simulink model "jaka_fk_exp"  (R2022b)
settings: Solver=FixedStepAuto  StartTime=0.0  StopTime=10.0  RelTol=1e-3
model workspace (MAT data in the model file):
  SL_ROS_VariableLengthArrays_MaxSizes.CommonInfo.ArrayTruncateAction = 'EmitWarning'
  SL_ROS_VariableLengthArrays_MaxSizes.MsgTypeMap = containers.Map
  SL_ROS_VariableLengthArrays_MaxSizes.MsgTypeMap.serialization.keys = {'jaka_msgs/MoveRequest'}
  SL_ROS_VariableLengthArrays_MaxSizes.MsgTypeMap.serialization.values{1}(1).PropertyName = 'Pose'
  SL_ROS_VariableLengthArrays_MaxSizes.MsgTypeMap.serialization.values{1}(1).DataType = 'single'
  SL_ROS_VariableLengthArrays_MaxSizes.MsgTypeMap.serialization.values{1}(1).MaxLength = 6
  SL_ROS_VariableLengthArrays_MaxSizes.MsgTypeMap.serialization.values{1}(2).PropertyName = 'RefJoint'
  SL_ROS_VariableLengthArrays_MaxSizes.MsgTypeMap.serialization.values{1}(2).DataType = 'single'
  SL_ROS_VariableLengthArrays_MaxSizes.MsgTypeMap.serialization.values{1}(2).MaxLength = 6
  SL_ROS_VariableLengthArrays_MaxSizes.MsgTypeMap.serialization.uniformity = 0
  SL_ROS_VariableLengthArrays_MaxSizes.MsgTypeMap.serialization.keyType = 'char'
  SL_ROS_VariableLengthArrays_MaxSizes.MsgTypeMap.serialization.valueType = 'any'
undefined symbols (not defined in the file or in its folder): Mvacc, Mvvelo, Pose, Pose_SL_Info
libraries: robotlib x2
settings Model: Creator=boen  LastModifiedBy=boen
settings OptimizationCC: EnhancedBackFolding=on  PassReuseOutputArgsAs=Individual arguments  ZeroExternalMemoryAtStartup=off  ZeroInternalMemoryAtStartup=off  MaxStackSize=64  OptimizeBlockOrder=speed  DifferentSizesBufferReuse=on  OptimizationCustomize=off  EfficientTunableParamExpr=on
settings DebuggingCC: ParameterTunabilityLossMsg=error
settings HardwareCC: ProdBitPerLong=64  ProdLargestAtomicInteger=LongLong  ProdLargestAtomicFloat=Double  ProdLongLongMode=on  ProdHWDeviceType=ARM Compatible->ARM 64-bit (LP64)
settings SFSimCC: MATLABDynamicMemAlloc=off
settings RTWCC: Description=Embedded Coder  SystemTargetFile=ert.tlc  HardwareBoard=Robot Operating System (ROS)  TLCOptions="-aInlineSetEventsForThisBaseRateFcn=TLC_FALSE -aSuppressMultiTaskScheduler=TLC_FALSE  -aRateBasedStepFcn=0"  TemplateMakefile=ert_default_tmf  Toolchain=Catkin  TargetLang=C++
settings CodeAppCC: ForceParamTrailComments=on  IgnoreCustomStorageClasses=off  OperatorAnnotations=on  SimulinkDataObjDesc=on  SFDataObjDesc=on  InsertBlockDesc=on

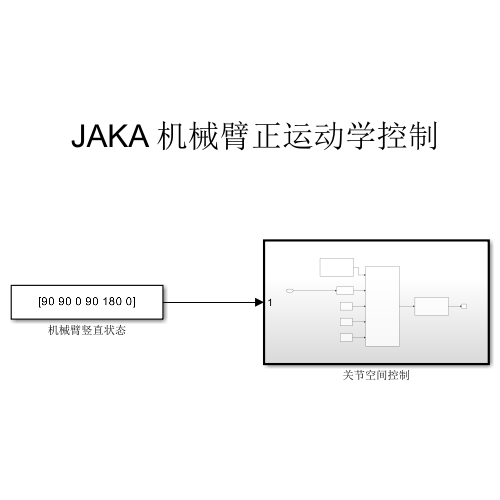
[thumbnail: Simulink's stored preview of the top-level diagram]
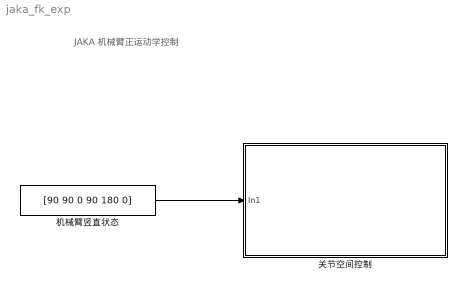
== system jaka_fk_exp ==
  note: JAKA 机械臂正运动学控制
  关节空间控制 : Subsystem  TreatAsAtomicUnit=on
  机械臂竖直状态 : Constant  Value=[90 90 0 90 180 0]
  wires:
  机械臂竖直状态/1 -> 关节空间控制/1(In1)

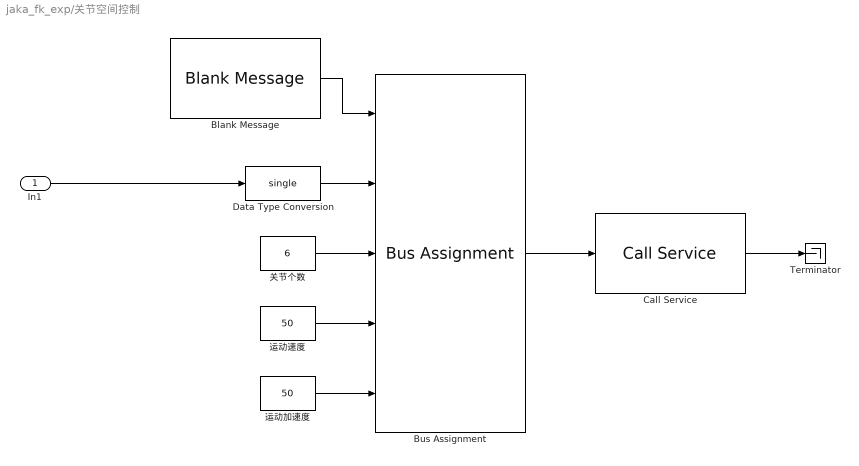
== system jaka_fk_exp/关节空间控制 ==
  In1 : Inport
  Blank Message : robotlib/Blank Message  messageClass=Service Request  entityType=jaka_msgs/Move  messageType=jaka_msgs/MoveRequest  SampleTime=inf  legacyBusStruct=off
  Bus Assignment : BusAssignment  AssignedSignals=Pose,Pose_SL_Info.CurrentLength,Mvacc,Mvvelo
  Call Service : robotlib/Call Service  topicSource=Select from ROS network  service=/robot_driver/move_joint  serviceType=jaka_msgs/Move  connectionTimeout=5  keepPersistent=off  ShowErrorCodeOutput=off  legacyBusStruct=off
  Data Type Conversion : DataTypeConversion  OutDataTypeStr=single  SaturateOnIntegerOverflow=off  RndMeth=Floor
  Terminator : Terminator
  关节个数 : Constant  Value=6  OutDataTypeStr=uint32
  运动加速度 : Constant  Value=50  OutDataTypeStr=single
  运动速度 : Constant  Value=50  OutDataTypeStr=single
  wires:
  Call Service/1 -> Terminator/1
  运动加速度/1 -> Bus Assignment/5
  Data Type Conversion/1 -> Bus Assignment/2
  Blank Message/1 -> Bus Assignment/1
  运动速度/1 -> Bus Assignment/4
  关节个数/1 -> Bus Assignment/3
  Bus Assignment/1 -> Call Service/1
  In1/1 -> Data Type Conversion/1
